simulink model "vdynblksskidpad_final"  (R2026b)
settings: Solver=ode23t  StopTime=inf  RelTol=5e-3
model workspace (MAT data in the model file):
  Eng : object (value not decoded)
  Nmtr = 11.5
  StartupTrim : object (value not decoded)
  SteerLim = 60
  TrackPoints = [-15 -12 -9 -6 -3 5.58745102111e-16 2.81978007367 5.36354042717 7.38228007367 8.67839071119 9.125 8.67839071119 ... (270 elements, 90x3)]
  Trans : object (value not decoded)
  Ts = 0.02
  VEH : object (value not decoded)
values from neighbouring files (symbols this model uses):
  n = size(e.Data,2)    [plot_skidpad_signals.m]
  z = tsMatrix(out.diagWheel.z)    [skidpad_settle_start.m]
symbols that are objects in the model workspace (value not decoded): Eng, StartupTrim, Trans, VEH
undefined symbols (not defined in the file or in its folder): BdyFrm, InertFrm, magnitude
libraries: autolibsharedcoupling x11, simulink x8, sim3dlib x7, autolibshareddiff x5, autolibutils x4, sim3dautolib x3, vehdynlibtirecommon x3, sharedtransform x3, vehdynlibdriver x2, vehdynlibsteering x2, vehdynlibeom x2, vehdynlibviscommon x2
(part 5 of 5)

== system vdynblksskidpad_final/Visualization/3D Visualization/Enabled/3D Visualization/Ground Following/Annotations/Enabled/Determine Angles In UE Vehicle Body Frame ==
  WheelYaw : Inport
  Fx : Inport  Port=2
  Fy : Inport  Port=3
  Add : Sum
  Add1 : Sum
  Constant1 : Constant  Value=0
  Constant11 : Constant  Value=[zeros(4,1)]
  Constant12 : Constant  Value=[zeros(4,1); ones(4,1).*pi/2]
  Constant2 : Constant  Value=pi
  Constant3 : Constant  Value=[zeros(8,2)]
  Constant4 : Constant  Value=[zeros(12,2)]
  Constant6 : Constant  Value=repmat([0 pi/2 0],[4,1])
  Matrix Concatenate : Concatenate  Mode=Multidimensional array
  Matrix Concatenate1 : Concatenate  Mode=Multidimensional array  ConcatenateDimension=2
  Matrix Concatenate2 : Concatenate  Mode=Multidimensional array
  Matrix Concatenate3 : Concatenate  NumInputs=3  Mode=Multidimensional array
  Matrix Concatenate4 : Concatenate  Mode=Multidimensional array  ConcatenateDimension=2
  Switch8 : Switch  ZeroCross=off  SaturateOnIntegerOverflow=off  InputSameDT=off
  Rotation : Outport
  wires:
  Constant2/1 -> Switch8/1
  Matrix Concatenate2/1 -> Switch8/2
  Constant1/1 -> Switch8/3
  Constant3/1 -> Matrix Concatenate1/1
  Matrix Concatenate1/1 -> Matrix Concatenate/1
  Switch8/1 -> Add/1
  Constant6/1 -> Matrix Concatenate/2
  Fx/1 -> Matrix Concatenate2/1
  Fy/1 -> Matrix Concatenate2/2
  Add/1 -> Matrix Concatenate1/2
  Constant12/1 -> Add/2
  Constant11/1 -> Matrix Concatenate3/3
  WheelYaw/1 -> Matrix Concatenate3/1, Matrix Concatenate3/2
  Constant4/1 -> Matrix Concatenate4/1
  Matrix Concatenate3/1 -> Matrix Concatenate4/2
  Matrix Concatenate4/1 -> Add1/2
  Matrix Concatenate/1 -> Add1/1
  Add1/1 -> Rotation/1

== system vdynblksskidpad_final/Visualization/3D Visualization/Enabled/3D Visualization/Physical Vehicle/Annotations/Enabled/Convert to string ==
  xdot : Inport
  MotorSpeed : Inport  Port=2
  Gear : Inport  Port=3
  Round : Rounding  Operator=round
  Round1 : Rounding  Operator=round
  Signal Specification : SignalSpecification  Unit=rpm
  Signal Specification1 : SignalSpecification  Unit=km/h
  String Concatenate1 : StringConcatenate  Inputs=3
  String Concatenate2 : StringConcatenate
  String Concatenate3 : StringConcatenate
  String Constant3 : StringConstant  String="\" km/h\\n\""
  String Constant4 : StringConstant  String="\" RPM\\n\""
  To String1 : ToString
  To String2 : ToString
  To String3 : ToString
  Unit Conversion : UnitConversion
  Unit Conversion1 : UnitConversion
  String : Outport
  wires:
  MotorSpeed/1 -> Unit Conversion/1
  Signal Specification/1 -> Round1/1
  String Constant4/1 -> String Concatenate3/2
  Signal Specification1/1 -> Round/1
  String Concatenate2/1 -> String Concatenate1/1
  To String2/1 -> String Concatenate2/1
  String Constant3/1 -> String Concatenate2/2
  To String1/1 -> String Concatenate1/3
  String Concatenate3/1 -> String Concatenate1/2
  To String3/1 -> String Concatenate3/1
  Round/1 -> To String2/1
  Round1/1 -> To String3/1
  String Concatenate1/1 -> String/1
  Gear/1 -> To String1/1
  Unit Conversion/1 -> Signal Specification/1
  Unit Conversion1/1 -> Signal Specification1/1
  xdot/1 -> Unit Conversion1/1

== system vdynblksskidpad_final/Visualization/3D Visualization/Enabled/3D Visualization/Physical Vehicle/Annotations/Enabled/Determine Angles In UE Vehicle Body Frame ==
  WheelYaw : Inport
  Fx : Inport  Port=2
  Fy : Inport  Port=3
  Add : Sum
  Add1 : Sum
  Constant1 : Constant  Value=0
  Constant11 : Constant  Value=[zeros(4,1)]
  Constant12 : Constant  Value=[zeros(4,1); ones(4,1).*pi/2]
  Constant2 : Constant  Value=pi
  Constant3 : Constant  Value=[zeros(8,2)]
  Constant4 : Constant  Value=[zeros(12,2)]
  Constant6 : Constant  Value=repmat([0 pi/2 0],[4,1])
  Matrix Concatenate : Concatenate  Mode=Multidimensional array
  Matrix Concatenate1 : Concatenate  Mode=Multidimensional array  ConcatenateDimension=2
  Matrix Concatenate2 : Concatenate  Mode=Multidimensional array
  Matrix Concatenate3 : Concatenate  NumInputs=3  Mode=Multidimensional array
  Matrix Concatenate4 : Concatenate  Mode=Multidimensional array  ConcatenateDimension=2
  Switch8 : Switch  ZeroCross=off  SaturateOnIntegerOverflow=off  InputSameDT=off
  Rotation : Outport
  wires:
  Constant2/1 -> Switch8/1
  Matrix Concatenate2/1 -> Switch8/2
  Constant1/1 -> Switch8/3
  Constant3/1 -> Matrix Concatenate1/1
  Matrix Concatenate1/1 -> Matrix Concatenate/1
  Switch8/1 -> Add/1
  Constant6/1 -> Matrix Concatenate/2
  Fx/1 -> Matrix Concatenate2/1
  Fy/1 -> Matrix Concatenate2/2
  Add/1 -> Matrix Concatenate1/2
  Constant12/1 -> Add/2
  Constant11/1 -> Matrix Concatenate3/3
  WheelYaw/1 -> Matrix Concatenate3/1, Matrix Concatenate3/2
  Constant4/1 -> Matrix Concatenate4/1
  Matrix Concatenate3/1 -> Matrix Concatenate4/2
  Matrix Concatenate4/1 -> Add1/2
  Matrix Concatenate/1 -> Add1/1
  Add1/1 -> Rotation/1

== system vdynblksskidpad_final/Visualization/3D Visualization/Enabled/3D Visualization/Simulation 3D Vehicle/Annotations/Enabled/Convert to string ==
  xdot : Inport
  MotorSpeed : Inport  Port=2
  Gear : Inport  Port=3
  Max : MinMax  Function=max  ZeroCross=off
  Round : Rounding  Operator=round
  Round1 : Rounding  Operator=round
  Signal Specification : SignalSpecification  Unit=rpm
  Signal Specification1 : SignalSpecification  Unit=km/h
  String Concatenate1 : StringConcatenate  Inputs=3
  String Concatenate2 : StringConcatenate
  String Concatenate3 : StringConcatenate
  String Constant3 : StringConstant  String="\" km/h\\n\""
  String Constant4 : StringConstant  String="\" RPM\\n\""
  To String1 : ToString
  To String2 : ToString
  To String3 : ToString
  Unit Conversion : UnitConversion
  Unit Conversion1 : UnitConversion
  String : Outport
  wires:
  MotorSpeed/1 -> Unit Conversion/1
  Signal Specification/1 -> Round1/1
  String Constant4/1 -> String Concatenate3/2
  Signal Specification1/1 -> Round/1
  String Concatenate2/1 -> String Concatenate1/1
  To String2/1 -> String Concatenate2/1
  String Constant3/1 -> String Concatenate2/2
  To String1/1 -> String Concatenate1/3
  String Concatenate3/1 -> String Concatenate1/2
  To String3/1 -> String Concatenate3/1
  Round/1 -> To String2/1
  Round1/1 -> Max/1
  String Concatenate1/1 -> String/1
  Gear/1 -> To String1/1
  Unit Conversion/1 -> Signal Specification/1
  Unit Conversion1/1 -> Signal Specification1/1
  xdot/1 -> Unit Conversion1/1
  Max/1 -> To String3/1

== system vdynblksskidpad_final/Visualization/3D Visualization/Enabled/3D Visualization/Simulation 3D Vehicle/Annotations/Enabled/Determine Angles In UE Vehicle Body Frame ==
  WheelYaw : Inport
  Fx : Inport  Port=2
  Fy : Inport  Port=3
  Add : Sum
  Add1 : Sum
  Constant1 : Constant  Value=0
  Constant11 : Constant  Value=[zeros(4,1)]
  Constant12 : Constant  Value=[zeros(4,1); ones(4,1).*pi/2]
  Constant2 : Constant  Value=pi
  Constant3 : Constant  Value=[zeros(8,2)]
  Constant4 : Constant  Value=[zeros(12,2)]
  Constant6 : Constant  Value=repmat([0 pi/2 0],[4,1])
  Matrix Concatenate : Concatenate  Mode=Multidimensional array
  Matrix Concatenate1 : Concatenate  Mode=Multidimensional array  ConcatenateDimension=2
  Matrix Concatenate2 : Concatenate  Mode=Multidimensional array
  Matrix Concatenate3 : Concatenate  NumInputs=3  Mode=Multidimensional array
  Matrix Concatenate4 : Concatenate  Mode=Multidimensional array  ConcatenateDimension=2
  Switch8 : Switch  ZeroCross=off  SaturateOnIntegerOverflow=off  InputSameDT=off
  Rotation : Outport
  wires:
  Constant2/1 -> Switch8/1
  Matrix Concatenate2/1 -> Switch8/2
  Constant1/1 -> Switch8/3
  Constant3/1 -> Matrix Concatenate1/1
  Matrix Concatenate1/1 -> Matrix Concatenate/1
  Switch8/1 -> Add/1
  Constant6/1 -> Matrix Concatenate/2
  Fx/1 -> Matrix Concatenate2/1
  Fy/1 -> Matrix Concatenate2/2
  Add/1 -> Matrix Concatenate1/2
  Constant12/1 -> Add/2
  Constant11/1 -> Matrix Concatenate3/3
  WheelYaw/1 -> Matrix Concatenate3/1, Matrix Concatenate3/2
  Constant4/1 -> Matrix Concatenate4/1
  Matrix Concatenate3/1 -> Matrix Concatenate4/2
  Matrix Concatenate4/1 -> Add1/2
  Matrix Concatenate/1 -> Add1/1
  Add1/1 -> Rotation/1

== matlab function vdynblksskidpad_final/Formula Student Vehicle/Simulink Physics - 7DOF/Powertrain & Driveline/Powertrain/4EM Powertrain/Torque Management ==
  data: Acc input; HndWhl input; MtrTrqCmd output; r input
function MtrTrqCmd = trqmngr(Acc, HndWhl, r)
Tmax = 5;
rmax = 500*pi/180;
Kr = 15;
MtrTrqCmd = ones(4,1).*Acc;
MtrTrqCmd(1:2) = 0;  % ← KILL FRONT MOTORS: RWD only
yawDiff = HndWhl - r./rmax;
MtrTrqCmd = (MtrTrqCmd +[1 -1 1 -1]'.*Kr.*yawDiff).*Tmax;
MtrTrqCmd(1:2) = 0;  % ← RE-ZERO after vectoring calc (so vectoring doesn't sneak torque to front)
maxTinds = abs(MtrTrqCmd)>Tmax;
MtrTrqCmd(maxTinds) = Tmax.*sign(MtrTrqCmd(maxTinds));

== matlab function vdynblksskidpad_final/Skidpad Reference/Lap Time Counter ==
  settings: updateMethod=DISCRETE
  data: X input; LapTimes output; Y input; psi input; t input; CurrLapNum output
function [LapTimes, CurrLapNum]  = laptimer(X, Y, psi, t)
% A very simple lap counter. Assumes the start line is at X = 0, along Y
% axis within a specified track width
%
% Copyright 2022 The MathWorks, Inc.
%
%#codegen
coder.allowpcode('plain')
NLaps = 4;
trackWidth = 3.5; 
[LapTimes, CurrLapNum] = vdynlaptimer(X, Y, psi, t,NLaps,trackWidth);
end
